simulink model "MotorFaultSystem"  (R2026a)
settings: Solver=FixedStepDiscrete  StopTime=7.9999  FixedStep=1/12000
settings Model: Creator=Tejashri  LastModifiedBy=Tejashri

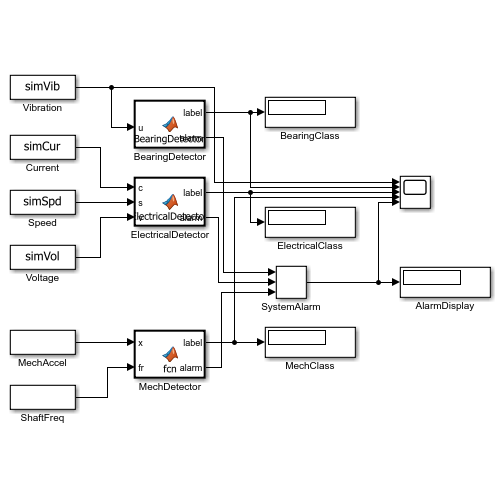
[thumbnail: Simulink's stored preview of the top-level diagram]
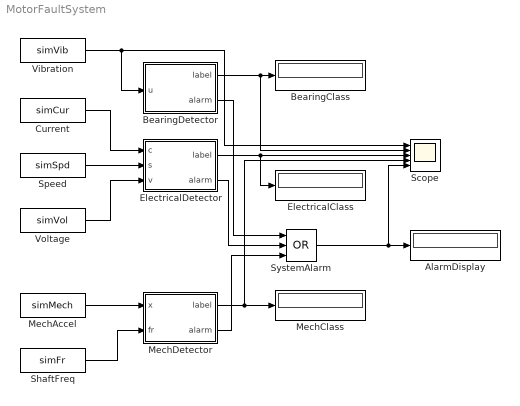
== system MotorFaultSystem ==
  AlarmDisplay : Display
  BearingClass : Display
  BearingDetector : MATLAB Function  TreatAsAtomicUnit=on
  Current : FromWorkspace  VariableName=simCur  SampleTime=1/12000  OutputAfterFinalValue=Holding final value
  ElectricalClass : Display
  ElectricalDetector : MATLAB Function  TreatAsAtomicUnit=on
  MechAccel : FromWorkspace  VariableName=simMech  SampleTime=1/12000  OutputAfterFinalValue=Holding final value
  MechClass : Display
  MechDetector : MATLAB Function  TreatAsAtomicUnit=on
  Scope : Scope  NumInputPorts=5
  ShaftFreq : FromWorkspace  VariableName=simFr  SampleTime=1/12000  OutputAfterFinalValue=Holding final value
  Speed : FromWorkspace  VariableName=simSpd  SampleTime=1/12000  OutputAfterFinalValue=Holding final value
  SystemAlarm : Logic  Operator=OR  Inputs=3  AllPortsSameDT=off  OutDataTypeStr=boolean
  Vibration : FromWorkspace  VariableName=simVib  SampleTime=1/12000  OutputAfterFinalValue=Holding final value
  Voltage : FromWorkspace  VariableName=simVol  SampleTime=1/12000  OutputAfterFinalValue=Holding final value
  wires:
  Vibration/1 -> Scope/1, BearingDetector/1(u)
  Current/1 -> ElectricalDetector/1(c)
  Speed/1 -> ElectricalDetector/2(s)
  Voltage/1 -> ElectricalDetector/3(v)
  MechAccel/1 -> MechDetector/1(x)
  ShaftFreq/1 -> MechDetector/2(fr)
  BearingDetector/2(alarm) -> SystemAlarm/1
  BearingDetector/1(label) -> Scope/2, BearingClass/1
  ElectricalDetector/1(label) -> Scope/3, ElectricalClass/1
  ElectricalDetector/2(alarm) -> SystemAlarm/2
  MechDetector/1(label) -> Scope/4, MechClass/1
  MechDetector/2(alarm) -> SystemAlarm/3
  SystemAlarm/1 -> Scope/5, AlarmDisplay/1

== matlab function MotorFaultSystem/ElectricalDetector ==
  data: c input; label output; s input; v input; alarm output
function [label, alarm] = ElectricalDetector(c, s, v)
[label, alarm] = electricalDetector(c, s, v);

== matlab function MotorFaultSystem/BearingDetector ==
  data: u input; label output; alarm output
function [label, alarm] = BearingDetector(u)
[label, alarm] = motorDetector(u);

== matlab function MotorFaultSystem/MechDetector ==
  data: x input; label output; fr input; alarm output
function [label, alarm] = MechDetector(x, fr)
[label, alarm] = mechanicalDetector(x, fr);
